simulink model "Trigger_CarrierPWM 1"  (R2022b)
settings: Solver=VariableStepAuto  StartTime=0.0  StopTime=1  RelTol=1e-3
libraries: spsGroundLib x1, spsPermanentMagnetSynchronousMachineLib x1, spsUniversalBridgeLib x1, spsDCVoltageSourceLib x1, sps_lib x1
settings Model: Creator=CSMotor  LastModifiedBy=CSMotor

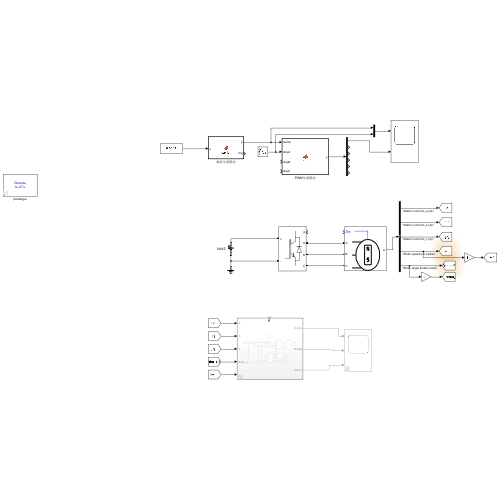
[thumbnail: Simulink's stored preview of the top-level diagram]
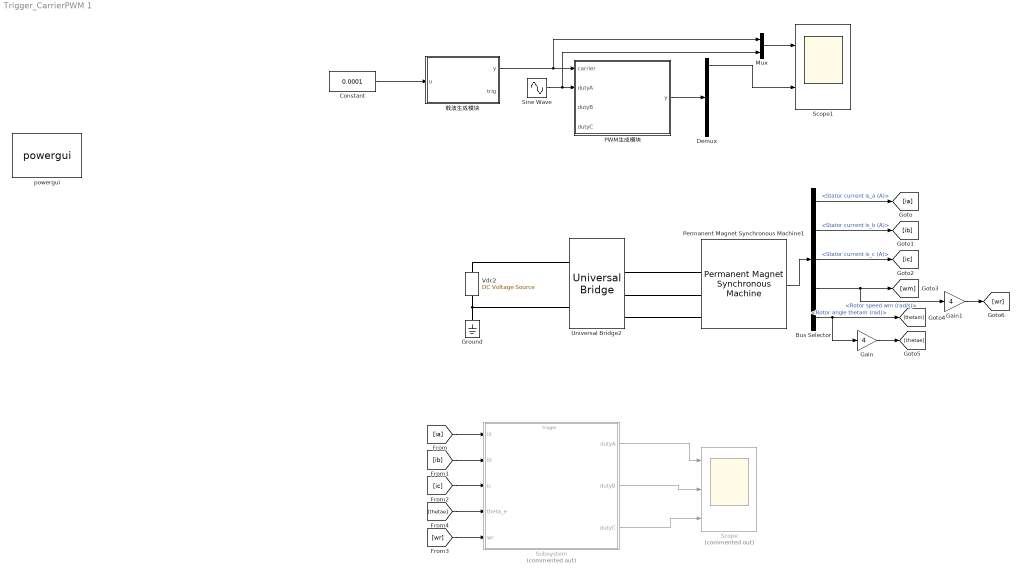
== system Trigger_CarrierPWM 1 ==
  Bus Selector : BusSelector  OutputSignals=Stator current is_a (A),Stator current is_b (A),Stator current is_c (A),Rotor speed wm (rad/s),Rotor angle thetam (rad)
  Constant : Constant  Value=0.0001
  Demux : Demux  Outputs=6
  Gain : Gain  Gain=4
  Gain1 : Gain  Gain=4
  Ground : spsGroundLib/Ground  LConnTagsString=a
  Mux : Mux  Inputs=2
  PWM生成模块 : MATLAB Function  TreatAsAtomicUnit=on
  Permanent Magnet Synchronous Machine1 : spsPermanentMagnetSynchronousMachineLib/Permanent Magnet Synchronous Machine  NbPhases=3  FluxDistribution=Sinusoidal  RotorType=Salient-pole  MechanicalLoad=Torque Tm  PresetModel="05:  8 Nm 300 Vdc 2000 RPM - 10 Nm"  ShowDetailedParameters=on  MeasurementBus=off  Resistance=0.9585  Inductance=8.5e-3  dqInductances=[0.004987 0.005513]  La=0.000835  MachineConstant=Flux linkage established by magnets (V.s)  Flux=0.1827  VoltageCst=132.5525  TorqueCst=1.0962  Flat=120  Mechanical=[0.0006329 0.0003035 4 0]  PolePairs=4  InitialConditions=[0,0, 0,0]  InitialConditions5ph=[0 0 0 0 0 0]  RefAngle=Aligned with phase A axis (original Park)  IterativeDiscreteModel=Trapezoidal non iterative  TsBlock=-1  TsPowergui=0
  Scope : Scope  Commented=on  NumInputPorts=3
  Scope1 : Scope  NumInputPorts=2
  Sine Wave : Sin  Amplitude=0.2  Bias=0.5  Frequency=50*2*pi  SampleTime=0
  Subsystem : Subsystem  Commented=on
  Universal Bridge2 : spsUniversalBridgeLib/Universal Bridge  Arms=3  SnubberResistance=1e5  SnubberCapacitance=inf  Device=IGBT / Diodes  Ron=1e-3  Lon=0  ForwardVoltages="[  0  0  ]"  ForwardVoltage=0  GTOparameters=[ 10e-6 , 20e-6 ]  IGBTparameters=[ 1e-6 , 2e-6 ]  Measurements=None  Measurements_2=None  converterType=Rectifier
  Vdc2 : spsDCVoltageSourceLib/DC Voltage Source  Amplitude=300  Measurements=None
  powergui : sps_lib/powergui  Priority=1  SimulationMode=Discrete  SampleTime=1e-7  frequency=60  Iterations=50  frequencyindice=0  Pbase=100e6  ErrMax=1e-4  UnitsV=kV  UnitsW=MW  buscounter=0  FunctionMessages=off  echomessages=off  EnableUseOfTLC=off  CurrentSourceSwitches=off  DisableSnubberDevices=off  DisableRonSwitches=off  DisableVfSwitches=off  DisplayEquations=off  AutomaticDiscreteSolvers=off  SolverType=Tustin/Backward Euler (TBE)  Interpol=off  ExternalGateDelay=off  methode=off  Ts=100  x0status=blocks  SPID=on  SwTol=0  HookPort=off  NonlinearTolerance=1e-4  nMaxIteration=100  ContinueOnMaxIteration=off  RestoreLinks=warning  ResistiveCurrentMeasurement=off  Frange=[0:2:500]  Ylog=off  Xlog=on  ShowGrid=off  save=off  variable=ZData  structure=0  ZoomFFT=off  StartTime=0.0  cycles=1  DisplayStyle=1  fundamental=60  FreqAxis=off  MaxFrequency=1000  frequencyindicesteady=1  RmsSteady=1  display=off
  载波生成模块 : MATLAB Function  TreatAsAtomicUnit=on
  wires:
  Subsystem/1(dutyA) -> Scope/1
  Subsystem/2(dutyB) -> Scope/2
  Subsystem/3(dutyC) -> Scope/3
  Constant/1 -> 载波生成模块/1(u)
  载波生成模块/1(y) -> Mux/1, PWM生成模块/1(carrier)
  Sine Wave/1 -> Mux/2, PWM生成模块/2(dutyA)
  PWM生成模块/1(y) -> Demux/1
  Mux/1 -> Scope1/1
  Demux/1 -> Scope1/2
  Permanent Magnet Synchronous Machine1/1 -> Bus Selector/1
  Bus Selector/1 -> [ia]  "<Stator current is_a (A)>"
  Bus Selector/2 -> [ib]  "<Stator current is_b (A)>"
  Bus Selector/3 -> [ic]  "<Stator current is_c (A)>"
  Bus Selector/4 -> Gain1/1, [wm]  "<Rotor speed wm (rad/s)>"
  Bus Selector/5 -> Gain/1, [thetam]  "<Rotor angle thetam (rad)>"
  Gain/1 -> [thetae]
  Gain1/1 -> [wr]
  [ia] -> Subsystem/1(ia)
  [ib] -> Subsystem/2(ib)
  [ic] -> Subsystem/3(ic)
  [wr] -> Subsystem/5(wr)
  [thetae] -> Subsystem/4(theta_e)
  connections:
  Permanent Magnet Synchronous Machine1/LConn1 -- Universal Bridge2/LConn1
  Permanent Magnet Synchronous Machine1/LConn2 -- Universal Bridge2/LConn2
  Permanent Magnet Synchronous Machine1/LConn3 -- Universal Bridge2/LConn3
  Vdc2/RConn1 -- Universal Bridge2/RConn1
  Vdc2/LConn1 -- Ground/LConn1 -- Universal Bridge2/RConn2

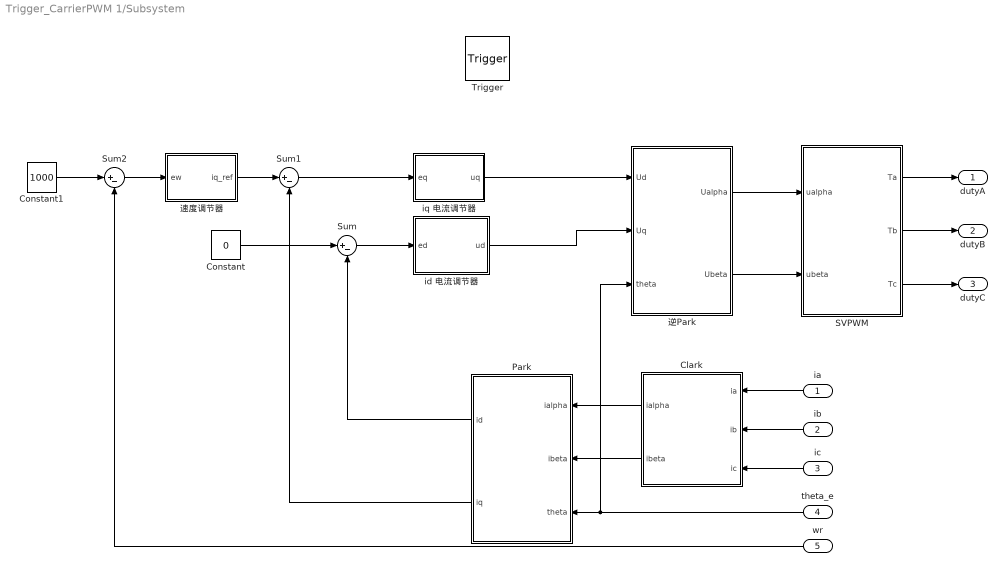
== system Trigger_CarrierPWM 1/Subsystem ==
  ia : Inport
  ib : Inport  Port=2
  ic : Inport  Port=3
  theta_e : Inport  Port=4
  wr : Inport  Port=5
  Trigger : TriggerPort  VariantControl=(inherit)  PortDimensions=1
  Clark : MATLAB Function  TreatAsAtomicUnit=on
  Constant : Constant  Value=0
  Constant1 : Constant  Value=1000
  Park : MATLAB Function  TreatAsAtomicUnit=on
  SVPWM : MATLAB Function  TreatAsAtomicUnit=on
  Sum : Sum  Inputs=|+-
  Sum1 : Sum  Inputs=|+-
  Sum2 : Sum  Inputs=|+-
  id 电流调节器 : MATLAB Function  TreatAsAtomicUnit=on
  iq 电流调节器 : MATLAB Function  TreatAsAtomicUnit=on
  逆Park : MATLAB Function  TreatAsAtomicUnit=on
  速度调节器 : MATLAB Function  TreatAsAtomicUnit=on
  dutyA : Outport
  dutyB : Outport  Port=2
  dutyC : Outport  Port=3
  wires:
  ia/1 -> Clark/1(ia)
  ib/1 -> Clark/2(ib)
  ic/1 -> Clark/3(ic)
  theta_e/1 -> 逆Park/3(theta), Park/3(theta)
  Clark/1(ialpha) -> Park/1(ialpha)
  Clark/2(ibeta) -> Park/2(ibeta)
  Park/1(id) -> Sum/2
  Sum/1 -> id 电流调节器/1(ed)
  Sum1/1 -> iq 电流调节器/1(eq)
  Park/2(iq) -> Sum1/2
  Constant/1 -> Sum/1
  速度调节器/1(iq_ref) -> Sum1/1
  iq 电流调节器/1(uq) -> 逆Park/1(Ud)
  id 电流调节器/1(ud) -> 逆Park/2(Uq)
  逆Park/1(Ualpha) -> SVPWM/1(ualpha)
  逆Park/2(Ubeta) -> SVPWM/2(ubeta)
  Sum2/1 -> 速度调节器/1(ew)
  wr/1 -> Sum2/2
  Constant1/1 -> Sum2/1
  SVPWM/1(Ta) -> dutyA/1
  SVPWM/2(Tb) -> dutyB/1
  SVPWM/3(Tc) -> dutyC/1

== matlab function Trigger_CarrierPWM 1/Subsystem/Clark ==
  data: ia input; ialpha output; ib input; ic input; ibeta output
function [ialpha, ibeta] = fcn(ia, ib, ic)
%#codegen
ialpha = (2/3) * (ia - 0.5*ib - 0.5*ic);
ibeta  = (2/3) * (sqrt(3)/2*ib - sqrt(3)/2*ic);

== matlab function Trigger_CarrierPWM 1/Subsystem/Park ==
  data: ialpha input; id output; ibeta input; theta input; iq output
function [id, iq] = fcn(ialpha, ibeta, theta)
%#codegen
id =  ialpha*cos(theta) + ibeta*sin(theta);
iq = -ialpha*sin(theta) + ibeta*cos(theta);

== matlab function Trigger_CarrierPWM 1/Subsystem/id 电流调节器 ==
  data: ed input; ud output
function ud = fcn_d(ed)
%#codegen
Ld = 0.004987;
Rs = 0.9585;
Ts = 0.0001;
Udc = 300;

Kp = Ld/(3*Ts);
Ki = Rs/(3*Ts);
Umax = Udc/sqrt(3);
int_lim = Umax/Ki;

persistent int_d
if isempty(int_d)
    int_d = 0;
end

int_d = int_d + ed*Ts;

if int_d >  int_lim, int_d =  int_lim; end
if int_d < -int_lim, int_d = -int_lim; end

ud = Kp*ed + Ki*int_d;

if ud >  Umax, ud =  Umax; end
if ud < -Umax, ud = -Umax; end

== matlab function Trigger_CarrierPWM 1/Subsystem/iq 电流调节器 ==
  data: eq input; uq output
function uq = fcn_q(eq)
%#codegen
Lq = 0.005513;
Rs = 0.9585;
Ts = 0.0001;
Udc = 300;

Kp = Lq/(3*Ts);
Ki = Rs/(3*Ts);
Umax = Udc/sqrt(3);
int_lim = Umax/Ki;

persistent int_q
if isempty(int_q)
    int_q = 0;
end

int_q = int_q + eq*Ts;

if int_q >  int_lim, int_q =  int_lim; end
if int_q < -int_lim, int_q = -int_lim; end

uq = Kp*eq + Ki*int_q;

if uq >  Umax, uq =  Umax; end
if uq < -Umax, uq = -Umax; end

== matlab function Trigger_CarrierPWM 1/Subsystem/速度调节器 ==
  data: ew input; iq_ref output
function iq_ref = fcn_w(ew)
%#codegen
Kp = 0.15;
Ki = 10;
Ts = 0.0001;

Imax    = 10;
int_lim = Imax/Ki;

persistent int_w
if isempty(int_w)
    int_w = 0;
end

int_w = int_w + ew*Ts;

if int_w >  int_lim, int_w =  int_lim; end
if int_w < -int_lim, int_w = -int_lim; end

iq_ref = Kp*ew + Ki*int_w;

if iq_ref >  Imax, iq_ref =  Imax; end
if iq_ref < -Imax, iq_ref = -Imax; end

== matlab function Trigger_CarrierPWM 1/Subsystem/逆Park ==
  data: Ud input; Ualpha output; Uq input; theta input; Ubeta output
function [Ualpha,Ubeta] = fcn(Ud, Uq, theta)
%#codegen
persistent acc
if isempty(acc)
    acc = 0;
end
acc = acc + step;
y = acc;

== matlab function Trigger_CarrierPWM 1/Subsystem/SVPWM ==
  data: ualpha input; Ta output; ubeta input; Tb output; Tc output
function [Ta, Tb, Tc] = fcn_svpwm(ualpha, ubeta)
%#codegen
SQRT3     = 1.73205080757;
SQRT3_INV = 0.57735026919;
Udc  = 300;

volAlphaNorm = ualpha/Udc*SQRT3;
volBetaNorm  = ubeta /Udc*SQRT3;

voltU = volAlphaNorm;
voltV = -0.5*volAlphaNorm + SQRT3*0.5*volBetaNorm;
voltW = -0.5*volAlphaNorm - SQRT3*0.5*volBetaNorm;

voltMax = max([voltU, voltV, voltW]);
voltMin = min([voltU, voltV, voltW]);
voltZero = -0.5*(voltMax + voltMin);

dutyU = SQRT3_INV*(voltU + voltZero) + 0.5;
dutyV = SQRT3_INV*(voltV + voltZero) + 0.5;
dutyW = SQRT3_INV*(voltW + voltZero) + 0.5;

Ta = min(max(dutyU, 0), 1);
Tb = min(max(dutyV, 0), 1);
Tc = min(max(dutyW, 0), 1);

== matlab function Trigger_CarrierPWM 1/载波生成模块 ==
  data: u input; y output; trig output
function [y, trig] = carrier(u)
%#codegen
persistent cnt dir
if isempty(cnt)
    cnt = 0;
    dir = 1;
end
Tdis = 1e-7;
n  = round(u/Tdis);
nh = n/2;

y = cnt/nh;
trig = (cnt == nh);

cnt = cnt + dir;
if cnt >= nh
    cnt = nh;
    dir = -1;
elseif cnt <= 0
    cnt = 0;
    dir = 1;
end

== matlab function Trigger_CarrierPWM 1/PWM生成模块 ==
  data: carrier input; y output; dutyA input; dutyB input; dutyC input
function y = fcn(carrier, dutyA, dutyB, dutyC)
%#codegen
ref  = carrier;
CMPA = dutyA;
CMPB = dutyB;
CMPC = dutyC;

Ta1 = 0;  Ta2 = 0;
Tb1 = 0;  Tb2 = 0;
Tc1 = 0;  Tc2 = 0;

if ref <= CMPA
    Ta1 = 1;  Ta2 = 0;
else
    Ta1 = 0;  Ta2 = 1;
end

if ref <= CMPB
    Tb1 = 1;  Tb2 = 0;
else
    Tb1 = 0;  Tb2 = 1;
end

if ref <= CMPC
    Tc1 = 1;  Tc2 = 0;
else
    Tc1 = 0;  Tc2 = 1;
end

y = [Ta1; Ta2; Tb1; Tb2; Tc1; Tc2];
